simulink model "sl_driveline"  (R2019b)
settings: Solver=ode45  StartTime=0.0  StopTime=15.0  RelTol=1e-3  EnableMultiTasking=on
InitFcn:
  | if ~exist('x0')
  |   x0 = [5 5 0];
  |   msgbox(sprintf('x0 not defined in workspace, setting it to [%g %g %g]\n', x0));
  | end
  | if ~exist('L')
  |   L = [1 -2 4];
  |   msgbox(sprintf('L not defined in workspace, setting it to [%g %g %g]\n', L));
  | end
  | % clean up old vehicle icons
  | set(0, 'ShowHiddenHandles', 'on')
  | delete(findobj('Tag', 'vehicle'))
  | set(0, 'ShowHiddenHandles', 'off')
StopFcn:
  | % update the XY scope
  | set(0, 'ShowHiddenHandles', 'on')
  | fig = findobj('name', 'XY');
  | ax = findobj(fig, 'type', 'axes');
  | axes(ax)
  | grid on
  | hold on
  | plot_vehicle(x0, 'r', 'Tag', 'vehicle')
  | plot_homline(L, 'r--', 'Tag', 'vehicle')
  | hold off
  | set(0, 'ShowHiddenHandles', 'off')
libraries: roblocks x2, simulink x1
settings Model: Creator=pic  LastModifiedBy=corkep
settings SolverCC: ZeroCrossAlgorithm=Adaptive
settings DataIOCC: SaveFormat=Array  TimeSaveName=t  OutputSaveName=y
settings OptimizationCC: ExpressionDepthLimit=2147483647  LifeSpan=inf
settings DebuggingCC: UnderspecifiedInitializationDetection=Classic  MergeDetectMultiDrivingBlocksExec=none  SolverPrmCheckMsg=warning  AllowSymbolicDim=off  StateNameClashWarn=warning  PregeneratedLibrarySubsystemCodeDiagnostic=none  SFUnexpectedBacktrackingDiag=warning  SFNoUnconditionalDefaultTransitionDiag=warning  SFExecutionAtInitializationDiag=none  ArithmeticOperatorsInVariantConditions=warning
settings HardwareCC: ProdBitPerPointer=32  ProdBitPerSizeT=32  ProdBitPerPtrDiffT=32  ProdLargestAtomicFloat=None  ProdIntDivRoundTo=Undefined  ProdEndianess=Unspecified  ProdWordSize=32  ProdHWDeviceType=32-bit Generic
settings ModelReferenceCC: PropagateSignalLabelsOutOfModel=off
settings SFSimCC: SimUseLocalCustomCode=off  CustomCodeUndefinedFunction=UseInterfaceOnly
settings RTWCC: RTWUseLocalCustomCode=off
settings CodeAppCC: StateflowObjectComments=on
settings GRTTargetCC: TargetLangStandard=C89/C90 (ANSI)  GeneratePreprocessorConditionals=Disable all  CombineOutputUpdateFcns=off  GRTInterface=on
settings ConfigComp: CovMetricSettings=dw  CovHtmlReporting=on  CovSaveCumulativeToWorkspaceVar=on  CovSaveSingleToWorkspaceVar=on  CovExternalEMLEnable=off

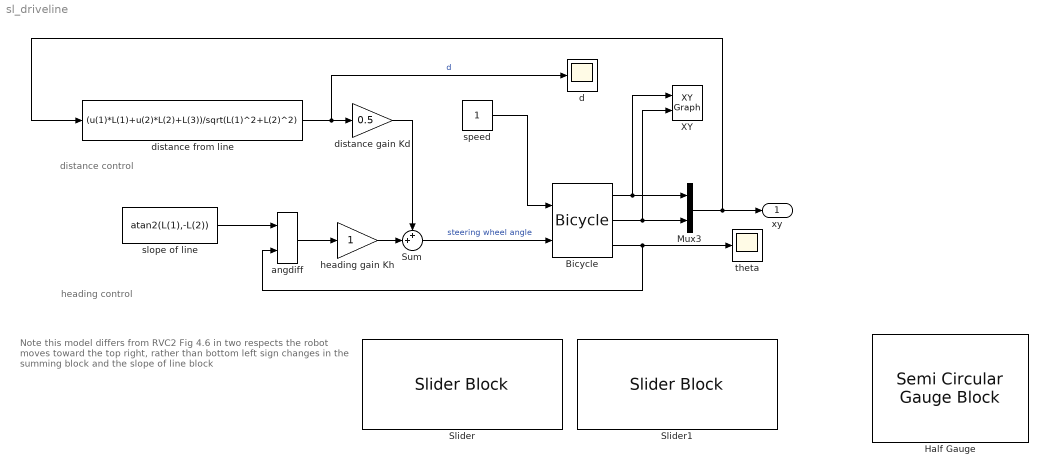
== system sl_driveline ==
  note: Note this model differs from RVC2 Fig 4.6 in two respects
      | the robot moves toward the top right, rather than bottom left
      | sign changes in the summing block and the slope of line block
  note: distance control
  note: heading control
  Bicycle : roblocks/Vehicles/Bicycle  vlim=1  accel=1  alim=1  steer_rate=Inf  L=1  x0=x0
  Half Gauge : SemiCircularGaugeBlock  LabelPosition=Bottom  ScaleMin=-1  ScaleMax=1
  Mux3 : Mux  Inputs=2
  Slider : SliderBlock  LabelPosition=Bottom  ScaleMax=1
  Slider1 : SliderBlock  LabelPosition=Bottom  ScaleMax=2
  Sum : Sum  Inputs=++|
  XY : simulink/Sinks/XY Graph  xmin=-10  xmax=10  ymin=-10  ymax=10  st=-1
  angdiff : roblocks/Toolbox/angdiff
  d : Scope
  distance from line : Fcn  Expr=(u(1)*L(1)+u(2)*L(2)+L(3))/sqrt(L(1)^2+L(2)^2)
  distance gain Kd : Gain  Gain=0.5
  heading gain Kh : Gain
  slope of line : Constant  Value=atan2(L(1),-L(2))
  speed : Constant  VectorParams1D=off  SampleTime=0.02
  theta : Scope
  xy : Outport  VectorParamsAs1DForOutWhenUnconnected=off
  wires:
  Mux3/1 -> distance from line/1, xy/1
  slope of line/1 -> angdiff/1
  angdiff/1 -> heading gain Kh/1
  heading gain Kh/1 -> Sum/2
  speed/1 -> Bicycle/1
  Sum/1 -> Bicycle/2  "steering wheel angle"
  distance from line/1 -> distance gain Kd/1, d/1  "d"
  Bicycle/1 -> XY/1, Mux3/1
  Bicycle/2 -> XY/2, Mux3/2
  Bicycle/3 -> angdiff/2, theta/1
  distance gain Kd/1 -> Sum/1
